simulink model "tank_model_open_loop"  (R2023b)
settings: Solver=VariableStepAuto  StartTime=0.0  StopTime=150  RelTol=1e-3
values from neighbouring files (symbols this model uses):
  c2_0 = 5.81    [tank_model.m]
  c3_0 = 4.48    [tank_model.m]
  h1_0 = 2.68    [tank_model.m]
  h2_0 = 1.85    [tank_model.m]
  h3_0 = 0.85    [tank_model.m]
  ua0 = 0.5    [tank_model.m]
  ud0 = 0.18    [tank_model.m]
  ur0 = 0.02    [tank_model.m]
undefined symbols (not defined in the file or in its folder): params
settings Model: Creator=fyder9  LastModifiedBy=fyder9

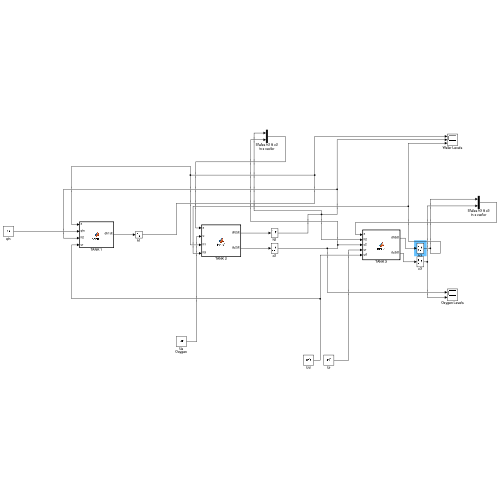
[thumbnail: Simulink's stored preview of the top-level diagram]
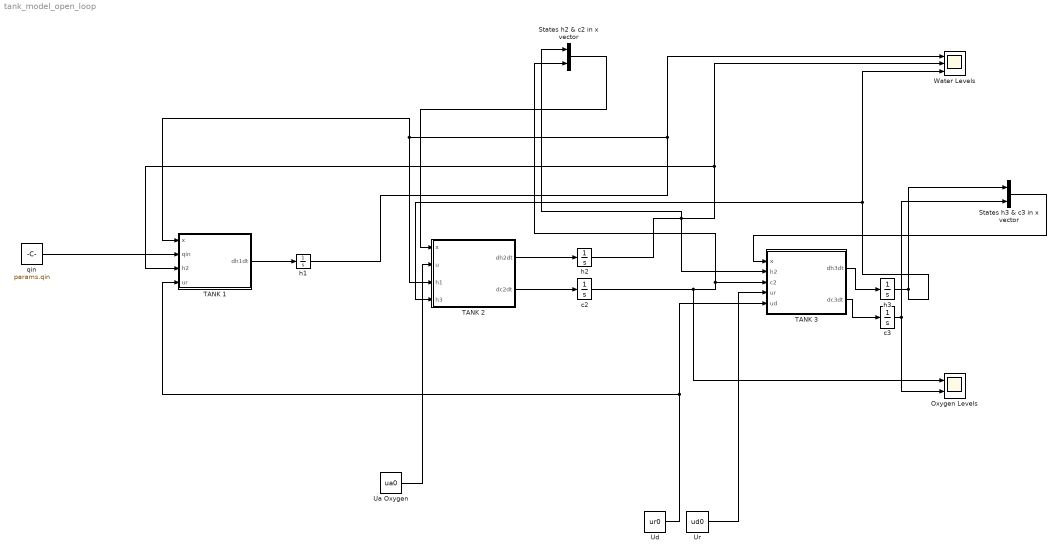
== system tank_model_open_loop ==
  Oxygen Levels : Scope  NumInputPorts=2
  States h2 & c2 in x vector : Mux  Inputs=2
  States h3 & c3 in x vector : Mux  Inputs=2
  TANK 1 : MATLAB Function  TreatAsAtomicUnit=on
  TANK 2 : MATLAB Function  TreatAsAtomicUnit=on
  TANK 3 : MATLAB Function  TreatAsAtomicUnit=on
  Ua Oxygen : Constant  Value=ua0
  Ud : Constant  Value=ur0
  Ur : Constant  Value=ud0
  Water Levels : Scope  NumInputPorts=3
  c2 : Integrator  InitialCondition=c2_0  LimitOutput=on  UpperSaturationLimit=8.0  LowerSaturationLimit=0
  c3 : Integrator  InitialCondition=c3_0  LimitOutput=on  UpperSaturationLimit=8.0  LowerSaturationLimit=0
  h1 : Integrator  InitialCondition=h1_0  LimitOutput=on  LowerSaturationLimit=0
  h2 : Integrator  InitialCondition=h2_0  LimitOutput=on  LowerSaturationLimit=0
  h3 : Integrator  InitialCondition=h3_0  LimitOutput=on  LowerSaturationLimit=0
  qin : Constant  Value=params.qin
  wires:
  TANK 2/1(dh2dt) -> h2/1
  h2/1 -> Water Levels/2, TANK 1/3(h2), TANK 3/2(h2), States h2 & c2 in x vector/1
  TANK 1/1(dh1dt) -> h1/1
  h1/1 -> Water Levels/1, TANK 2/3(h1), TANK 1/1(x)
  qin/1 -> TANK 1/2(qin)
  TANK 2/2(dc2dt) -> c2/1
  c2/1 -> Oxygen Levels/1, States h2 & c2 in x vector/2, TANK 3/3(c2)
  States h2 & c2 in x vector/1 -> TANK 2/1(x)
  Ua Oxygen/1 -> TANK 2/2(u)
  TANK 3/1(dh3dt) -> h3/1
  h3/1 -> Water Levels/3, TANK 2/4(h3), States h3 & c3 in x vector/1
  TANK 3/2(dc3dt) -> c3/1
  c3/1 -> Oxygen Levels/2, States h3 & c3 in x vector/2
  States h3 & c3 in x vector/1 -> TANK 3/1(x)
  Ur/1 -> TANK 3/4(ur)
  Ud/1 -> TANK 3/5(ud), TANK 1/4(ur)

== matlab function tank_model_open_loop/TANK 2 ==
  data: x input; u input; dh2dt output size=1; h1 input; h3 input; dc2dt output size=1
function [dh2dt, dc2dt] = tank2(x, u, h1, h3)

%states
h2 = max(x(1), 1e-3);
c2 = max(x(2), 0);
%params
A1 = 1.2;
A2 = 1.0;
cin = 1.0;
k12 = 0.22;
k23 = 0.20;
csat = 8.0;
lambda2 = 0.08;
ka = 0.9;
%input
ua = u;
%flow
q12 = k12 * sqrt(max(h1 - h2, 0));
q23 = k23 * sqrt(max(h2 - h3, 0));
q12 = min(q12, h1*A1); 
q23 = min(q23, h2*A2);
%output
dh2dt = (q12 - q23)/A2;
dc2dt = (q12/(A2*h2) * (cin - c2) + ka*ua*(csat-c2)-lambda2*c2);
end

== matlab function tank_model_open_loop/TANK 1 ==
  data: x input; qin input; dh1dt output size=1; h2 input; ur input
function dh1dt = tank1(x, qin, h2, ur)
%state
h1 = max(x, 1e-3);
%params
A1 = 1.2;
cin = 1.0;
k12 = 0.22;
%input ur
%flow rate
q12 = k12 * sqrt(max(h1 - h2, 0));
q12 = min(q12, h1*A1);
dh1dt = ((qin + ur)-(q12))/A1;
end

== matlab function tank_model_open_loop/TANK 3 ==
  data: x input; dh3dt output size=1; h2 input; c2 input; dc3dt output size=1; ur input; ud input
function [dh3dt, dc3dt] = tank3(x, h2, c2, ur , ud)

%states
c3 = x(2);
h3 = max(x(1),1e-3);
%params
A2 = 1.0;
A3 = 1.4;
lambda3 = 0.05;
k23 = 0.20;
%flow
q23 = k23 * sqrt(max(h2 - h3, 0));
q23 = min(q23, h2*A2);
%output
dh3dt = (q23 - ud - ur)/A3;
dc3dt = (q23/(A3*h3)) * (c2 - c3) - lambda3*c3;

end
